simulink model "Pune_HVAC_BlockDiagram"  (R2024a)
settings: Solver=FixedStepDiscrete  StartTime=0.0  StopTime=(7*96-1)*SL.Ts  FixedStep=SL.Ts  RelTol=1e-3
values from neighbouring files (symbols this model uses):
  SL = sl_blocks('init', 'base', c, 1, n_days); assignin('base', 'SL', SL)    [check_simulink_model.m]    (also in sl_blocks.m = struct())
libraries: simulink x6
settings Model: Creator=deshm  LastModifiedBy=deshm
settings DataIOCC: SaveOutput=off
settings DebuggingCC: AlgebraicLoopMsg=error

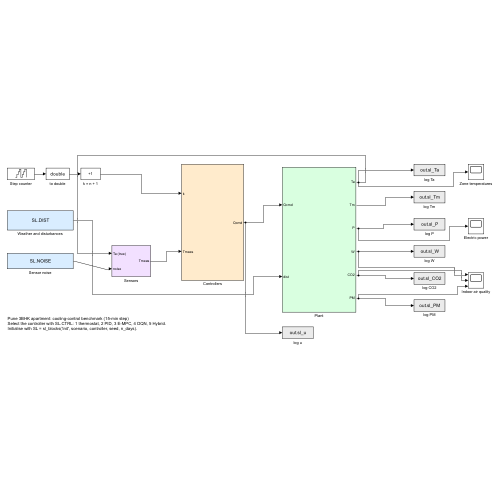
[thumbnail: Simulink's stored preview of the top-level diagram]
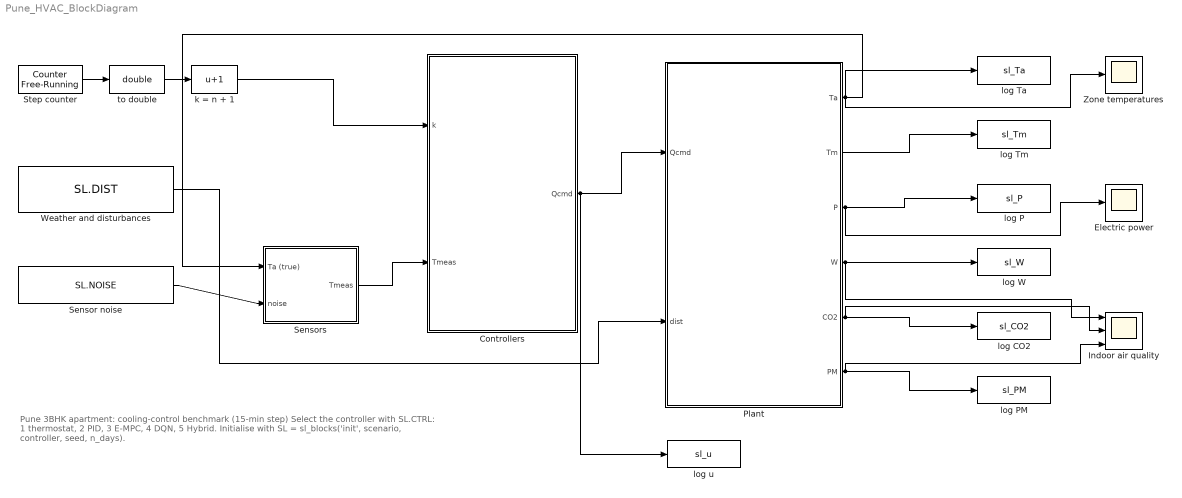
== system Pune_HVAC_BlockDiagram ==
  note: Pune 3BHK apartment: cooling-control benchmark (15-min step)
      | Select the controller with SL.CTRL: 1 thermostat, 2 PID, 3 E-MPC, 4 DQN, 5 Hybrid.
      | Initialise with SL = sl_blocks('init', scenario, controller, seed, n_days).
  Controllers : Subsystem
  Electric power : Scope
  Indoor air quality : Scope  NumInputPorts=3
  Plant : Subsystem
  Sensor noise : FromWorkspace  VariableName=SL.NOISE  SampleTime=SL.Ts  Interpolate=off  OutputAfterFinalValue=Holding final value
  Sensors : Subsystem
  Step counter : simulink/Sources/Counter Free-Running  NumBits=32  tsamp=SL.Ts
  Weather and disturbances : FromWorkspace  VariableName=SL.DIST  SampleTime=SL.Ts  Interpolate=off  OutputAfterFinalValue=Holding final value
  Zone temperatures : Scope
  k = n + 1 : Bias  Bias=1  SaturateOnIntegerOverflow=off
  log CO2 : ToWorkspace  VariableName=sl_CO2  SampleTime=SL.Ts
  log P : ToWorkspace  VariableName=sl_P  SampleTime=SL.Ts
  log PM : ToWorkspace  VariableName=sl_PM  SampleTime=SL.Ts
  log Ta : ToWorkspace  VariableName=sl_Ta  SampleTime=SL.Ts
  log Tm : ToWorkspace  VariableName=sl_Tm  SampleTime=SL.Ts
  log W : ToWorkspace  VariableName=sl_W  SampleTime=SL.Ts
  log u : ToWorkspace  VariableName=sl_u  SampleTime=SL.Ts
  to double : DataTypeConversion  OutDataTypeStr=double  SaturateOnIntegerOverflow=off  RndMeth=Floor
  wires:
  Step counter/1 -> to double/1
  to double/1 -> k = n + 1/1
  Sensor noise/1 -> Sensors/2(noise)
  k = n + 1/1 -> Controllers/1(k)
  Sensors/1(Tmeas) -> Controllers/2(Tmeas)
  Controllers/1(Qcmd) -> Plant/1(Qcmd), log u/1
  Weather and disturbances/1 -> Plant/2(dist)
  Plant/1(Ta) -> Sensors/1(Ta (true)), log Ta/1, Zone temperatures/1
  Plant/2(Tm) -> log Tm/1
  Plant/3(P) -> log P/1, Electric power/1
  Plant/4(W) -> log W/1, Indoor air quality/1
  Plant/5(CO2) -> log CO2/1, Indoor air quality/2
  Plant/6(PM) -> log PM/1, Indoor air quality/3

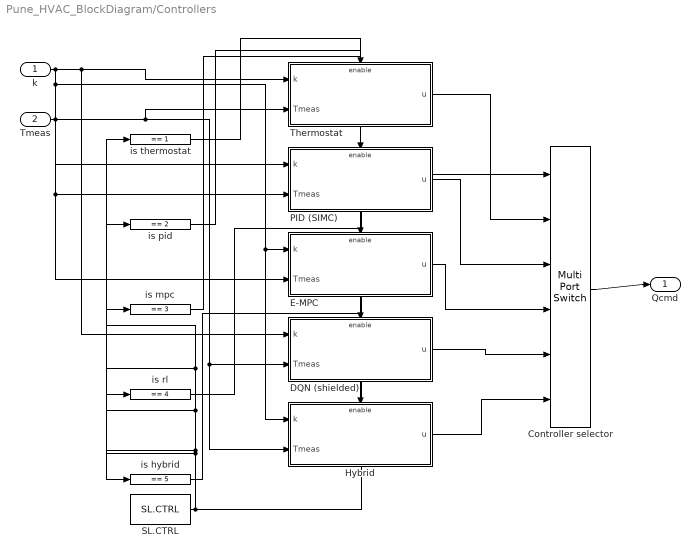
== system Pune_HVAC_BlockDiagram/Controllers ==
  k : Inport
  Tmeas : Inport  Port=2
  Controller selector : MultiPortSwitch  Inputs=5  SaturateOnIntegerOverflow=off  InputSameDT=off
  DQN (shielded) : Subsystem  TreatAsAtomicUnit=on
  E-MPC : Subsystem  TreatAsAtomicUnit=on
  Hybrid : Subsystem  TreatAsAtomicUnit=on
  PID (SIMC) : Subsystem  TreatAsAtomicUnit=on
  SL.CTRL : Constant  Value=SL.CTRL
  Thermostat : Subsystem  TreatAsAtomicUnit=on
  is hybrid : simulink/Logic and Bit Operations/Compare To Constant  relop===  const=5  OutDataTypeStr=boolean
  is mpc : simulink/Logic and Bit Operations/Compare To Constant  relop===  const=3  OutDataTypeStr=boolean
  is pid : simulink/Logic and Bit Operations/Compare To Constant  relop===  const=2  OutDataTypeStr=boolean
  is rl : simulink/Logic and Bit Operations/Compare To Constant  relop===  const=4  OutDataTypeStr=boolean
  is thermostat : simulink/Logic and Bit Operations/Compare To Constant  relop===  const=1  OutDataTypeStr=boolean
  Qcmd : Outport
  wires:
  SL.CTRL/1 -> is thermostat/1, is pid/1, is mpc/1, is hybrid/1, is rl/1, Controller selector/1
  is thermostat/1 -> Thermostat/Enable
  k/1 -> E-MPC/1(k), Hybrid/1(k), PID (SIMC)/1(k), Thermostat/1(k), DQN (shielded)/1(k)
  Tmeas/1 -> PID (SIMC)/2(Tmeas), E-MPC/2(Tmeas), DQN (shielded)/2(Tmeas), Hybrid/2(Tmeas), Thermostat/2(Tmeas)
  Thermostat/1(u) -> Controller selector/2
  is pid/1 -> PID (SIMC)/Enable
  PID (SIMC)/1(u) -> Controller selector/3
  is mpc/1 -> E-MPC/Enable
  E-MPC/1(u) -> Controller selector/4
  is rl/1 -> DQN (shielded)/Enable
  DQN (shielded)/1(u) -> Controller selector/5
  is hybrid/1 -> Hybrid/Enable
  Hybrid/1(u) -> Controller selector/6
  Controller selector/1 -> Qcmd/1

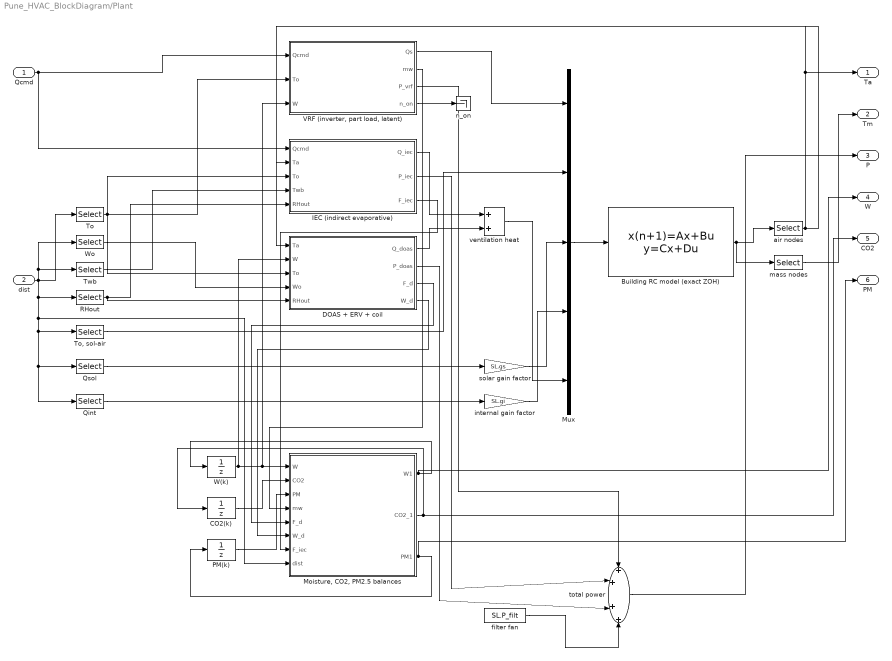
== system Pune_HVAC_BlockDiagram/Plant ==
  Qcmd : Inport
  dist : Inport  Port=2
  Building RC model (exact ZOH) : DiscreteStateSpace  A=SL.Ad  B=SL.B  C=eye(6)  D=zeros(6,17)  InitialCondition=SL.x0  SampleTime=SL.Ts
  CO2(k) : UnitDelay  InitialCondition=SL.CO2_0  SampleTime=SL.Ts  HasFrameUpgradeWarning=on
  DOAS + ERV + coil : MATLAB Function  TreatAsAtomicUnit=on
  IEC (indirect evaporative) : MATLAB Function  TreatAsAtomicUnit=on
  "Moisture, CO2, PM2.5 balances" : MATLAB Function  TreatAsAtomicUnit=on
  Mux : Mux  Inputs=5
  PM(k) : UnitDelay  InitialCondition=SL.PM0  SampleTime=SL.Ts  HasFrameUpgradeWarning=on
  Qint : Selector  IndexOptions=Index vector (dialog)  Indices=[12 13 14]  OutputSizes=1
  Qsol : Selector  IndexOptions=Index vector (dialog)  Indices=[9 10 11]  OutputSizes=1
  RHout : Selector  IndexOptions=Index vector (dialog)  Indices=4  OutputSizes=1
  To : Selector  IndexOptions=Index vector (dialog)  Indices=1  OutputSizes=1
  "To, sol-air" : Selector  IndexOptions=Index vector (dialog)  Indices=[1 5 6 7 8]  OutputSizes=1
  Twb : Selector  IndexOptions=Index vector (dialog)  Indices=3  OutputSizes=1
  "VRF (inverter, part load, latent)" : MATLAB Function  TreatAsAtomicUnit=on
  W(k) : UnitDelay  InitialCondition=SL.W0  SampleTime=SL.Ts  HasFrameUpgradeWarning=on
  Wo : Selector  IndexOptions=Index vector (dialog)  Indices=2  OutputSizes=1
  air nodes : Selector  IndexOptions=Index vector (dialog)  Indices=1:3  OutputSizes=1
  filter fan : Constant  Value=SL.P_filt
  internal gain factor : Gain  Gain=SL.gi
  mass nodes : Selector  IndexOptions=Index vector (dialog)  Indices=4:6  OutputSizes=1
  n_on : Terminator
  solar gain factor : Gain  Gain=SL.gs
  total power : Sum  Inputs=++++
  ventilation heat : Sum
  Ta : Outport
  Tm : Outport  Port=2
  P : Outport  Port=3
  W : Outport  Port=4
  CO2 : Outport  Port=5
  PM : Outport  Port=6
  wires:
  dist/1 -> Qsol/1, Qint/1, "To, sol-air"/1, "Moisture, CO2, PM2.5 balances"/8(dist), RHout/1, Wo/1, Twb/1, To/1
  Qcmd/1 -> "VRF (inverter, part load, latent)"/1(Qcmd), IEC (indirect evaporative)/1(Qcmd)
  To/1 -> "VRF (inverter, part load, latent)"/2(To), IEC (indirect evaporative)/3(To), DOAS + ERV + coil/3(To)
  W(k)/1 -> "VRF (inverter, part load, latent)"/3(W), "Moisture, CO2, PM2.5 balances"/1(W), DOAS + ERV + coil/2(W)
  air nodes/1 -> DOAS + ERV + coil/1(Ta), Ta/1, IEC (indirect evaporative)/2(Ta)
  Twb/1 -> IEC (indirect evaporative)/4(Twb)
  RHout/1 -> IEC (indirect evaporative)/5(RHout), DOAS + ERV + coil/5(RHout)
  Wo/1 -> DOAS + ERV + coil/4(Wo)
  "VRF (inverter, part load, latent)"/1(Qs) -> Mux/1
  "To, sol-air"/1 -> Mux/2
  Qsol/1 -> solar gain factor/1
  solar gain factor/1 -> Mux/3
  Qint/1 -> internal gain factor/1
  internal gain factor/1 -> Mux/4
  IEC (indirect evaporative)/1(Q_iec) -> ventilation heat/1
  DOAS + ERV + coil/1(Q_doas) -> ventilation heat/2
  ventilation heat/1 -> Mux/5
  Mux/1 -> Building RC model (exact ZOH)/1
  Building RC model (exact ZOH)/1 -> air nodes/1, mass nodes/1
  CO2(k)/1 -> "Moisture, CO2, PM2.5 balances"/2(CO2)
  PM(k)/1 -> "Moisture, CO2, PM2.5 balances"/3(PM)
  "VRF (inverter, part load, latent)"/2(mw) -> "Moisture, CO2, PM2.5 balances"/4(mw)
  DOAS + ERV + coil/3(F_d) -> "Moisture, CO2, PM2.5 balances"/5(F_d)
  DOAS + ERV + coil/4(W_d) -> "Moisture, CO2, PM2.5 balances"/6(W_d)
  IEC (indirect evaporative)/3(F_iec) -> "Moisture, CO2, PM2.5 balances"/7(F_iec)
  "Moisture, CO2, PM2.5 balances"/1(W1) -> W(k)/1, W/1
  "Moisture, CO2, PM2.5 balances"/2(CO2_1) -> CO2(k)/1, CO2/1
  "Moisture, CO2, PM2.5 balances"/3(PM1) -> PM(k)/1, PM/1
  "VRF (inverter, part load, latent)"/3(P_vrf) -> total power/1
  IEC (indirect evaporative)/2(P_iec) -> total power/2
  DOAS + ERV + coil/2(P_doas) -> total power/3
  filter fan/1 -> total power/4
  mass nodes/1 -> Tm/1
  total power/1 -> P/1
  "VRF (inverter, part load, latent)"/4(n_on) -> n_on/1

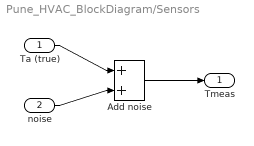
== system Pune_HVAC_BlockDiagram/Sensors ==
  Ta (true) : Inport
  noise : Inport  Port=2
  Add noise : Sum
  Tmeas : Outport
  wires:
  Ta (true)/1 -> Add noise/1
  noise/1 -> Add noise/2
  Add noise/1 -> Tmeas/1

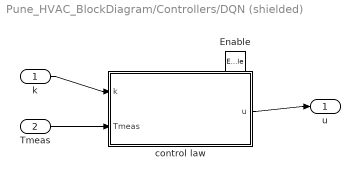
== system Pune_HVAC_BlockDiagram/Controllers/DQN (shielded) ==
  k : Inport
  Tmeas : Inport  Port=2
  Enable : EnablePort
  control law : MATLAB Function  TreatAsAtomicUnit=on
  u : Outport
  wires:
  k/1 -> control law/1(k)
  Tmeas/1 -> control law/2(Tmeas)
  control law/1(u) -> u/1

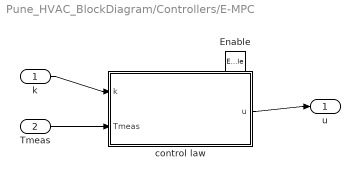
== system Pune_HVAC_BlockDiagram/Controllers/E-MPC ==
  k : Inport
  Tmeas : Inport  Port=2
  Enable : EnablePort
  control law : MATLAB Function  TreatAsAtomicUnit=on
  u : Outport
  wires:
  k/1 -> control law/1(k)
  Tmeas/1 -> control law/2(Tmeas)
  control law/1(u) -> u/1

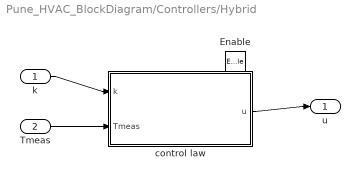
== system Pune_HVAC_BlockDiagram/Controllers/Hybrid ==
  k : Inport
  Tmeas : Inport  Port=2
  Enable : EnablePort
  control law : MATLAB Function  TreatAsAtomicUnit=on
  u : Outport
  wires:
  k/1 -> control law/1(k)
  Tmeas/1 -> control law/2(Tmeas)
  control law/1(u) -> u/1

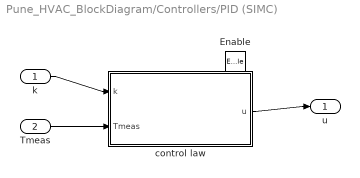
== system Pune_HVAC_BlockDiagram/Controllers/PID (SIMC) ==
  k : Inport
  Tmeas : Inport  Port=2
  Enable : EnablePort
  control law : MATLAB Function  TreatAsAtomicUnit=on
  u : Outport
  wires:
  k/1 -> control law/1(k)
  Tmeas/1 -> control law/2(Tmeas)
  control law/1(u) -> u/1

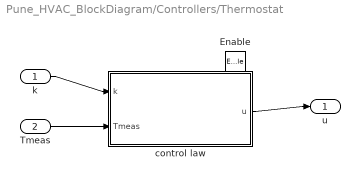
== system Pune_HVAC_BlockDiagram/Controllers/Thermostat ==
  k : Inport
  Tmeas : Inport  Port=2
  Enable : EnablePort
  control law : MATLAB Function  TreatAsAtomicUnit=on
  u : Outport
  wires:
  k/1 -> control law/1(k)
  Tmeas/1 -> control law/2(Tmeas)
  control law/1(u) -> u/1

== matlab function Pune_HVAC_BlockDiagram/Controllers/PID (SIMC)/control law ==
  data: k input; u output; Tmeas input
function u = control_law(k, Tmeas)
% PID (SIMC) controller (see src/controllers)
coder.extrinsic('sl_blocks');
u = zeros(3,1);
u = sl_blocks('ctrl', 'pid', k, Tmeas);

== matlab function Pune_HVAC_BlockDiagram/Controllers/Thermostat/control law ==
  data: k input; u output; Tmeas input
function u = control_law(k, Tmeas)
% Thermostat controller (see src/controllers)
coder.extrinsic('sl_blocks');
u = zeros(3,1);
u = sl_blocks('ctrl', 'thermostat', k, Tmeas);

== matlab function Pune_HVAC_BlockDiagram/Controllers/E-MPC/control law ==
  data: k input; u output; Tmeas input
function u = control_law(k, Tmeas)
% E-MPC controller (see src/controllers)
coder.extrinsic('sl_blocks');
u = zeros(3,1);
u = sl_blocks('ctrl', 'mpc', k, Tmeas);

== matlab function Pune_HVAC_BlockDiagram/Controllers/DQN (shielded)/control law ==
  data: k input; u output; Tmeas input
function u = control_law(k, Tmeas)
% DQN (shielded) controller (see src/controllers)
coder.extrinsic('sl_blocks');
u = zeros(3,1);
u = sl_blocks('ctrl', 'rl', k, Tmeas);

== matlab function Pune_HVAC_BlockDiagram/Controllers/Hybrid/control law ==
  data: k input; u output; Tmeas input
function u = control_law(k, Tmeas)
% Hybrid controller (see src/controllers)
coder.extrinsic('sl_blocks');
u = zeros(3,1);
u = sl_blocks('ctrl', 'hybrid', k, Tmeas);

== matlab function Pune_HVAC_BlockDiagram/Plant/VRF (inverter, part load, latent) ==
  data: Qcmd input; Qs output; To input; W input; mw output; P_vrf output; n_on output
function [Qs, mw, P_vrf, n_on] = vrf(Qcmd, To, W)
coder.extrinsic('sl_blocks');
Qs = zeros(3,1); mw = 0; P_vrf = 0; n_on = 0;
[Qs, mw, P_vrf, n_on] = sl_blocks('vrf', Qcmd, To, W);

== matlab function Pune_HVAC_BlockDiagram/Plant/IEC (indirect evaporative) ==
  data: Qcmd input; Q_iec output; Ta input; To input; Twb input; RHout input; P_iec output; F_iec output
function [Q_iec, P_iec, F_iec] = iec(Qcmd, Ta, To, Twb, RHout)
coder.extrinsic('sl_blocks');
Q_iec = zeros(3,1); P_iec = 0; F_iec = 0;
[Q_iec, P_iec, F_iec] = sl_blocks('iec', Qcmd, Ta, To, Twb, RHout);

== matlab function Pune_HVAC_BlockDiagram/Plant/DOAS + ERV + coil ==
  data: Ta input; Q_doas output; W input; To input; Wo input; RHout input; P_doas output; F_d output; W_d output
function [Q_doas, P_doas, F_d, W_d] = doas(Ta, W, To, Wo, RHout)
coder.extrinsic('sl_blocks');
Q_doas = zeros(3,1); P_doas = 0; F_d = 0; W_d = 0;
[Q_doas, P_doas, F_d, W_d] = sl_blocks('doas', Ta, W, To, Wo, RHout);

== matlab function Pune_HVAC_BlockDiagram/Plant/Moisture, CO2, PM2.5 balances ==
  data: W input; W1 output; CO2 input; PM input; mw input; F_d input; W_d input; F_iec input; dist input; CO2_1 output; PM1 output
function [W1, CO2_1, PM1] = iaq(W, CO2, PM, mw, F_d, W_d, F_iec, dist)
coder.extrinsic('sl_blocks');
W1 = 0; CO2_1 = 0; PM1 = 0;
[W1, CO2_1, PM1] = sl_blocks('iaq', W, CO2, PM, mw, F_d, W_d, F_iec, dist);
